simulink model "Main_SpeedOptimisedVersionTannenweg"  (R2024b)
settings: Solver=ode15s  StartTime=0.0  StopTime=3600*2  FixedStep=0.1  RelTol=0.001
model workspace (MAT data in the model file):
  Ti = 5
  fa = 0.00071
  fd = 0.03
  ips = 36
  ma = 0.0013
  md = 0.04
  roomarea1 = 20
  s = 15
libraries: fl_lib x1434, nesl_utility x105, SimscapeFluids_lib x35
(part 2 of 22)

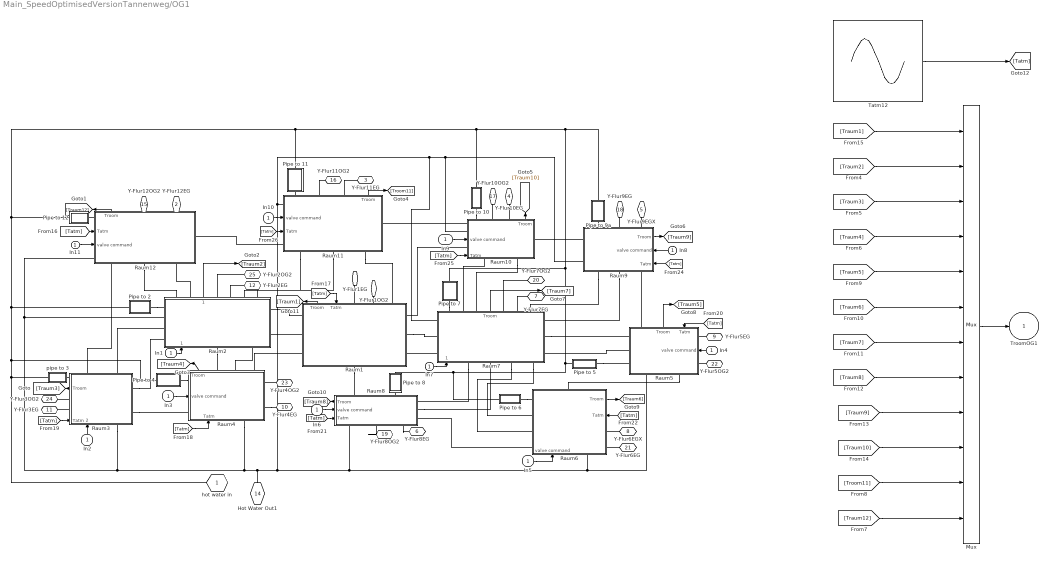
== system Main_SpeedOptimisedVersionTannenweg/OG1 ==
  In1 : Inport
  In{2..11} (10 alike) : InportShadow
  Mux : Mux  Inputs=12
  Pipe to 10 : Subsystem
  Pipe to 11 : Subsystem
  Pipe to 12 : Subsystem
  Pipe to 2 : Subsystem
  Pipe to 4 : Subsystem
  Pipe to 5 : Subsystem
  Pipe to 6 : Subsystem
  Pipe to 7 : Subsystem
  Pipe to 8 : Subsystem
  Pipe to 9a : Subsystem
  Raum1 : Subsystem
      settings: PortSchema="{\"entries\":[{\"content\":{\"sides\":[{\"content\":{\"connectorIds\":[\"LConn1\",\"LConn2\",\"LConn3\"]},\"type\":\"ConnectorPlacement.EquallySpacedRectSide\",\"uuid\":\"258852ae-79b4-4e90-ae22-4154c858ab0a\"},{\"content\":{\"connectorIds\":[\"RConn1\",\"RConn2\",\"RConn3\"],\"side\":\"RIGHT\"},\"type\":\"ConnectorPlacement.EquallySpacedRectSide\",\"uuid\":\"36706832-f330-42ce-9a32-f145cdee4912\"},{\"content\":{\"connectorIds\":[\"LConn4\",\"LConn5\",\"LConn6\",\"In1\",\"Out1\"],\"side\":\"TOP\"},\"type\":\"ConnectorPlacement.EquallySpacedRectSide\",\"uuid\":\"5cf2347a-3520-447e-9561-2d1c8313f3cf\"},{\"content\":{\"connectorIds\":[\"RConn4\"],\"side\":\"BOTTOM\"},\"type\":\"ConnectorPlacement.EquallySpacedRectSide\",\"uuid\":\"b1588268-8d41-4423-8f6e-2c28bf9b13dc\"}]},\"type\":\"ConnectorPlacement.EquallySpacedConnector\",\"uuid\":\"6bed35e7-1d7a-421b-a1f8-39267ed9017d\"}],\"packageUris\":[\"http://schema.mathworks.com/mf0/Connector/R2020b\"],\"version\":\"1.0\"}"
  Raum10 : Subsystem
      settings: PortSchema="{\"entries\":[{\"content\":{\"sides\":[{\"content\":{\"connectorIds\":[\"LConn1\",\"LConn2\",\"In1\",\"LConn3\",\"In2\"]},\"type\":\"ConnectorPlacement.EquallySpacedRectSide\",\"uuid\":\"258852ae-79b4-4e90-ae22-4154c858ab0a\"},{\"content\":{\"connectorIds\":[\"RConn1\"],\"side\":\"RIGHT\"},\"type\":\"ConnectorPlacement.EquallySpacedRectSide\",\"uuid\":\"36706832-f330-42ce-9a32-f145cdee4912\"},{\"content\":{\"connectorIds\":[\"LConn4\",\"LConn5\",\"LConn6\",\"Out1\"],\"side\":\"TOP\"},\"type\":\"ConnectorPlacement.EquallySpacedRectSide\",\"uuid\":\"5cf2347a-3520-447e-9561-2d1c8313f3cf\"},{\"content\":{\"connectorIds\":[\"RConn2\",\"RConn3\"],\"side\":\"BOTTOM\"},\"type\":\"ConnectorPlacement.EquallySpacedRectSide\",\"uuid\":\"b1588268-8d41-4423-8f6e-2c28bf9b13dc\"}]},\"type\":\"ConnectorPlacement.EquallySpacedConnector\",\"uuid\":\"6bed35e7-1d7a-421b-a1f8-39267ed9017d\"}],\"packageUris\":[\"http://schema.mathworks.com/mf0/Connector/R2020b\"],\"version\":\"1.0\"}"
  Raum11 : Subsystem
      settings: PortSchema="{\"entries\":[{\"content\":{\"sides\":[{\"content\":{\"connectorIds\":[\"LConn1\",\"In1\",\"In2\",\"LConn2\"]},\"type\":\"ConnectorPlacement.EquallySpacedRectSide\",\"uuid\":\"258852ae-79b4-4e90-ae22-4154c858ab0a\"},{\"content\":{\"connectorIds\":[\"RConn1\"],\"side\":\"RIGHT\"},\"type\":\"ConnectorPlacement.EquallySpacedRectSide\",\"uuid\":\"36706832-f330-42ce-9a32-f145cdee4912\"},{\"content\":{\"connectorIds\":[\"LConn3\",\"LConn4\",\"LConn5\",\"Out1\"],\"side\":\"TOP\"},\"type\":\"ConnectorPlacement.EquallySpacedRectSide\",\"uuid\":\"5cf2347a-3520-447e-9561-2d1c8313f3cf\"},{\"content\":{\"connectorIds\":[\"RConn2\",\"RConn3\",\"RConn4\"],\"side\":\"BOTTOM\"},\"type\":\"ConnectorPlacement.EquallySpacedRectSide\",\"uuid\":\"b1588268-8d41-4423-8f6e-2c28bf9b13dc\"}]},\"type\":\"ConnectorPlacement.EquallySpacedConnector\",\"uuid\":\"6bed35e7-1d7a-421b-a1f8-39267ed9017d\"}],\"packageUris\":[\"http://schema.mathworks.com/mf0/Connector/R2020b\"],\"version\":\"1.0\"}"
  Raum12 : Subsystem
      settings: PortSchema="{\"entries\":[{\"content\":{\"sides\":[{\"content\":{\"connectorIds\":[\"LConn1\",\"In1\",\"In2\",\"LConn2\"]},\"type\":\"ConnectorPlacement.EquallySpacedRectSide\",\"uuid\":\"258852ae-79b4-4e90-ae22-4154c858ab0a\"},{\"content\":{\"connectorIds\":[\"RConn1\"],\"side\":\"RIGHT\"},\"type\":\"ConnectorPlacement.EquallySpacedRectSide\",\"uuid\":\"36706832-f330-42ce-9a32-f145cdee4912\"},{\"content\":{\"connectorIds\":[\"Out1\",\"LConn3\",\"LConn4\"],\"side\":\"TOP\"},\"type\":\"ConnectorPlacement.EquallySpacedRectSide\",\"uuid\":\"5cf2347a-3520-447e-9561-2d1c8313f3cf\"},{\"content\":{\"connectorIds\":[\"RConn2\",\"RConn3\",\"RConn4\"],\"side\":\"BOTTOM\"},\"type\":\"ConnectorPlacement.EquallySpacedRectSide\",\"uuid\":\"b1588268-8d41-4423-8f6e-2c28bf9b13dc\"}]},\"type\":\"ConnectorPlacement.EquallySpacedConnector\",\"uuid\":\"6bed35e7-1d7a-421b-a1f8-39267ed9017d\"}],\"packageUris\":[\"http://schema.mathworks.com/mf0/Connector/R2020b\"],\"version\":\"1.0\"}"
  Raum2 : Subsystem
      settings: PortSchema="{\"entries\":[{\"content\":{\"sides\":[{\"content\":{\"connectorIds\":[\"LConn1\",\"LConn2\",\"LConn3\",\"LConn4\"]},\"type\":\"ConnectorPlacement.EquallySpacedRectSide\",\"uuid\":\"258852ae-79b4-4e90-ae22-4154c858ab0a\"},{\"content\":{\"connectorIds\":[\"RConn1\",\"RConn2\"],\"side\":\"RIGHT\"},\"type\":\"ConnectorPlacement.EquallySpacedRectSide\",\"uuid\":\"36706832-f330-42ce-9a32-f145cdee4912\"},{\"content\":{\"connectorIds\":[\"LConn5\",\"LConn6\",\"Out1\",\"LConn7\",\"LConn8\",\"LConn9\",\"LConn10\"],\"side\":\"TOP\"},\"type\":\"ConnectorPlacement.EquallySpacedRectSide\",\"uuid\":\"5cf2347a-3520-447e-9561-2d1c8313f3cf\"},{\"content\":{\"connectorIds\":[\"In1\",\"RConn3\",\"RConn4\"],\"side\":\"BOTTOM\"},\"type\":\"ConnectorPlacement.EquallySpacedRectSide\",\"uuid\":\"b1588268-8d41-4423-8f6e-2c28bf9b13dc\"}]},\"type\":\"ConnectorPlacement.EquallySpacedConnector\",\"uuid\":\"6bed35e7-1d7a-421b-a1f8-39267ed9017d\"}],\"packageUris\":[\"http://schema.mathworks.com/mf0/Connector/R2020b\"],\"version\":\"1.0\"}"
  Raum3 : Subsystem
      settings: PortSchema="{\"entries\":[{\"content\":{\"sides\":[{\"content\":{\"connectorIds\":[\"LConn1\",\"Out1\",\"LConn2\",\"LConn3\",\"In1\"]},\"type\":\"ConnectorPlacement.EquallySpacedRectSide\",\"uuid\":\"258852ae-79b4-4e90-ae22-4154c858ab0a\"},{\"content\":{\"connectorIds\":[\"RConn1\",\"RConn2\"],\"side\":\"RIGHT\"},\"type\":\"ConnectorPlacement.EquallySpacedRectSide\",\"uuid\":\"36706832-f330-42ce-9a32-f145cdee4912\"},{\"content\":{\"connectorIds\":[\"LConn4\",\"LConn5\"],\"side\":\"TOP\"},\"type\":\"ConnectorPlacement.EquallySpacedRectSide\",\"uuid\":\"5cf2347a-3520-447e-9561-2d1c8313f3cf\"},{\"content\":{\"connectorIds\":[\"In2\",\"RConn3\"],\"side\":\"BOTTOM\"},\"type\":\"ConnectorPlacement.EquallySpacedRectSide\",\"uuid\":\"b1588268-8d41-4423-8f6e-2c28bf9b13dc\"}]},\"type\":\"ConnectorPlacement.EquallySpacedConnector\",\"uuid\":\"6bed35e7-1d7a-421b-a1f8-39267ed9017d\"}],\"packageUris\":[\"http://schema.mathworks.com/mf0/Connector/R2020b\"],\"version\":\"1.0\"}"
  Raum4 : Subsystem
      settings: PortSchema="{\"entries\":[{\"content\":{\"sides\":[{\"content\":{\"connectorIds\":[\"LConn1\",\"In1\",\"LConn2\"]},\"type\":\"ConnectorPlacement.EquallySpacedRectSide\",\"uuid\":\"258852ae-79b4-4e90-ae22-4154c858ab0a\"},{\"content\":{\"connectorIds\":[\"RConn1\",\"RConn2\"],\"side\":\"RIGHT\"},\"type\":\"ConnectorPlacement.EquallySpacedRectSide\",\"uuid\":\"36706832-f330-42ce-9a32-f145cdee4912\"},{\"content\":{\"connectorIds\":[\"Out1\",\"LConn3\",\"LConn4\",\"LConn5\"],\"side\":\"TOP\"},\"type\":\"ConnectorPlacement.EquallySpacedRectSide\",\"uuid\":\"5cf2347a-3520-447e-9561-2d1c8313f3cf\"},{\"content\":{\"connectorIds\":[\"In2\",\"RConn3\"],\"side\":\"BOTTOM\"},\"type\":\"ConnectorPlacement.EquallySpacedRectSide\",\"uuid\":\"b1588268-8d41-4423-8f6e-2c28bf9b13dc\"}]},\"type\":\"ConnectorPlacement.EquallySpacedConnector\",\"uuid\":\"6bed35e7-1d7a-421b-a1f8-39267ed9017d\"}],\"packageUris\":[\"http://schema.mathworks.com/mf0/Connector/R2020b\"],\"version\":\"1.0\"}"
  Raum5 : Subsystem
      settings: PortSchema="{\"entries\":[{\"content\":{\"sides\":[{\"content\":{\"connectorIds\":[\"LConn1\",\"LConn2\",\"LConn3\"]},\"type\":\"ConnectorPlacement.EquallySpacedRectSide\",\"uuid\":\"258852ae-79b4-4e90-ae22-4154c858ab0a\"},{\"content\":{\"connectorIds\":[\"RConn1\",\"In2\",\"RConn2\"],\"side\":\"RIGHT\"},\"type\":\"ConnectorPlacement.EquallySpacedRectSide\",\"uuid\":\"36706832-f330-42ce-9a32-f145cdee4912\"},{\"content\":{\"connectorIds\":[\"LConn4\",\"Out1\",\"In1\"],\"side\":\"TOP\"},\"type\":\"ConnectorPlacement.EquallySpacedRectSide\",\"uuid\":\"5cf2347a-3520-447e-9561-2d1c8313f3cf\"},{\"content\":{\"connectorIds\":[\"RConn3\",\"RConn4\"],\"side\":\"BOTTOM\"},\"type\":\"ConnectorPlacement.EquallySpacedRectSide\",\"uuid\":\"b1588268-8d41-4423-8f6e-2c28bf9b13dc\"}]},\"type\":\"ConnectorPlacement.EquallySpacedConnector\",\"uuid\":\"6bed35e7-1d7a-421b-a1f8-39267ed9017d\"}],\"packageUris\":[\"http://schema.mathworks.com/mf0/Connector/R2020b\"],\"version\":\"1.0\"}"
  Raum6 : Subsystem
      settings: PortSchema="{\"entries\":[{\"content\":{\"sides\":[{\"content\":{\"connectorIds\":[\"LConn1\",\"LConn2\",\"LConn3\",\"LConn4\"]},\"type\":\"ConnectorPlacement.EquallySpacedRectSide\",\"uuid\":\"258852ae-79b4-4e90-ae22-4154c858ab0a\"},{\"content\":{\"connectorIds\":[\"Out1\",\"In2\",\"RConn1\",\"RConn2\"],\"side\":\"RIGHT\"},\"type\":\"ConnectorPlacement.EquallySpacedRectSide\",\"uuid\":\"36706832-f330-42ce-9a32-f145cdee4912\"},{\"content\":{\"connectorIds\":[\"LConn5\"],\"side\":\"TOP\"},\"type\":\"ConnectorPlacement.EquallySpacedRectSide\",\"uuid\":\"5cf2347a-3520-447e-9561-2d1c8313f3cf\"},{\"content\":{\"connectorIds\":[\"In1\",\"RConn3\"],\"side\":\"BOTTOM\"},\"type\":\"ConnectorPlacement.EquallySpacedRectSide\",\"uuid\":\"b1588268-8d41-4423-8f6e-2c28bf9b13dc\"}]},\"type\":\"ConnectorPlacement.EquallySpacedConnector\",\"uuid\":\"6bed35e7-1d7a-421b-a1f8-39267ed9017d\"}],\"packageUris\":[\"http://schema.mathworks.com/mf0/Connector/R2020b\"],\"version\":\"1.0\"}"
  Raum7 : Subsystem
      settings: PortSchema="{\"entries\":[{\"content\":{\"sides\":[{\"content\":{\"connectorIds\":[\"LConn1\",\"LConn2\",\"LConn3\"]},\"type\":\"ConnectorPlacement.EquallySpacedRectSide\",\"uuid\":\"258852ae-79b4-4e90-ae22-4154c858ab0a\"},{\"content\":{\"connectorIds\":[\"RConn1\",\"RConn2\",\"RConn3\"],\"side\":\"RIGHT\"},\"type\":\"ConnectorPlacement.EquallySpacedRectSide\",\"uuid\":\"36706832-f330-42ce-9a32-f145cdee4912\"},{\"content\":{\"connectorIds\":[\"LConn4\",\"LConn5\",\"LConn6\",\"Out1\",\"LConn7\",\"LConn8\",\"LConn9\"],\"side\":\"TOP\"},\"type\":\"ConnectorPlacement.EquallySpacedRectSide\",\"uuid\":\"5cf2347a-3520-447e-9561-2d1c8313f3cf\"},{\"content\":{\"connectorIds\":[\"In1\",\"RConn4\",\"RConn5\",\"RConn6\",\"RConn7\"],\"side\":\"BOTTOM\"},\"type\":\"ConnectorPlacement.EquallySpacedRectSide\",\"uuid\":\"b1588268-8d41-4423-8f6e-2c28bf9b13dc\"}]},\"type\":\"ConnectorPlacement.EquallySpacedConnector\",\"uuid\":\"6bed35e7-1d7a-421b-a1f8-39267ed9017d\"}],\"packageUris\":[\"http://schema.mathworks.com/mf0/Connector/R2020b\"],\"version\":\"1.0\"}"
  Raum8 : Subsystem
      settings: PortSchema="{\"entries\":[{\"content\":{\"sides\":[{\"content\":{\"connectorIds\":[\"Out1\",\"In1\",\"In2\"]},\"type\":\"ConnectorPlacement.EquallySpacedRectSide\",\"uuid\":\"258852ae-79b4-4e90-ae22-4154c858ab0a\"},{\"content\":{\"connectorIds\":[\"RConn1\",\"RConn2\",\"RConn3\"],\"side\":\"RIGHT\"},\"type\":\"ConnectorPlacement.EquallySpacedRectSide\",\"uuid\":\"36706832-f330-42ce-9a32-f145cdee4912\"},{\"content\":{\"connectorIds\":[\"LConn1\",\"LConn2\"],\"side\":\"TOP\"},\"type\":\"ConnectorPlacement.EquallySpacedRectSide\",\"uuid\":\"5cf2347a-3520-447e-9561-2d1c8313f3cf\"},{\"content\":{\"connectorIds\":[\"RConn4\",\"RConn5\",\"RConn6\"],\"side\":\"BOTTOM\"},\"type\":\"ConnectorPlacement.EquallySpacedRectSide\",\"uuid\":\"b1588268-8d41-4423-8f6e-2c28bf9b13dc\"}]},\"type\":\"ConnectorPlacement.EquallySpacedConnector\",\"uuid\":\"6bed35e7-1d7a-421b-a1f8-39267ed9017d\"}],\"packageUris\":[\"http://schema.mathworks.com/mf0/Connector/R2020b\"],\"version\":\"1.0\"}"
  Raum9 : Subsystem
      settings: PortSchema="{\"entries\":[{\"content\":{\"sides\":[{\"content\":{\"connectorIds\":[\"LConn1\",\"LConn2\"]},\"type\":\"ConnectorPlacement.EquallySpacedRectSide\",\"uuid\":\"258852ae-79b4-4e90-ae22-4154c858ab0a\"},{\"content\":{\"connectorIds\":[\"Out1\",\"In1\",\"In2\"],\"side\":\"RIGHT\"},\"type\":\"ConnectorPlacement.EquallySpacedRectSide\",\"uuid\":\"36706832-f330-42ce-9a32-f145cdee4912\"},{\"content\":{\"connectorIds\":[\"LConn3\",\"LConn4\",\"LConn5\"],\"side\":\"TOP\"},\"type\":\"ConnectorPlacement.EquallySpacedRectSide\",\"uuid\":\"5cf2347a-3520-447e-9561-2d1c8313f3cf\"},{\"content\":{\"connectorIds\":[\"RConn1\",\"RConn2\",\"RConn3\"],\"side\":\"BOTTOM\"},\"type\":\"ConnectorPlacement.EquallySpacedRectSide\",\"uuid\":\"b1588268-8d41-4423-8f6e-2c28bf9b13dc\"}]},\"type\":\"ConnectorPlacement.EquallySpacedConnector\",\"uuid\":\"6bed35e7-1d7a-421b-a1f8-39267ed9017d\"}],\"packageUris\":[\"http://schema.mathworks.com/mf0/Connector/R2020b\"],\"version\":\"1.0\"}"
  Tatm12 : Sin  Amplitude=7  Frequency=2*pi/(24*3600)  Phase=pi  SampleTime=0
  pipe to 3 : Subsystem
  hot water in : PMIOPort  Side=Left
  Y-Flur12EG : PMIOPort  Port=2  Side=Left
  Y-Flur11EG : PMIOPort  Port=3  Side=Left
  Y-Flur10EG : PMIOPort  Port=4  Side=Left
  Y-Flur9EGX : PMIOPort  Port=5  Side=Left
  Y-Flur8EG : PMIOPort  Port=6  Side=Left
  Y-Flur7EG : PMIOPort  Port=7  Side=Left
  Y-Flur6EGX : PMIOPort  Port=8  Side=Left
  Y-Flur5EG : PMIOPort  Port=9  Side=Left
  Y-Flur4EG : PMIOPort  Port=10  Side=Left
  Y-Flur3EG : PMIOPort  Port=11  Side=Left
  Y-Flur2EG : PMIOPort  Port=12  Side=Left
  Y-Flur1EG : PMIOPort  Port=13  Side=Left
  Hot Water Out1 : PMIOPort  Port=14  Side=Right
  Y-Flur12OG2 : PMIOPort  Port=15  Side=Right
  Y-Flur11OG2 : PMIOPort  Port=16  Side=Right
  Y-Flur10OG2 : PMIOPort  Port=17  Side=Right
  Y-Flur9EG : PMIOPort  Port=18  Side=Right
  Y-Flur8OG2 : PMIOPort  Port=19  Side=Right
  Y-Flur7OG2 : PMIOPort  Port=20  Side=Right
  Y-Flur6EG : PMIOPort  Port=21  Side=Right
  Y-Flur5OG2 : PMIOPort  Port=22  Side=Right
  Y-Flur4OG2 : PMIOPort  Port=23  Side=Right
  Y-Flur3OG2 : PMIOPort  Port=24  Side=Right
  Y-Flur2OG2 : PMIOPort  Port=25  Side=Right
  Y-Flur1OG2 : PMIOPort  Port=26  Side=Right
  TroomOG1 : Outport
  wires:
  [Tatm] -> Raum12/1(Tatm)
  Raum12/1(Troom) -> [Traum12]
  Raum8/1(Troom) -> [Traum8]
  Raum5/1(Troom) -> [Traum5]
  Raum4/1(Troom) -> [Traum4]
  [Tatm] -> Raum8/2(Tatm)
  [Tatm] -> Raum6/2(Tatm)
  Raum1/1(Troom) -> [Traum1]
  Raum10/1(Troom) -> [Traum10]
  Raum3/1(Troom) -> [Traum3]
  [Tatm] -> Raum4/2(Tatm)
  [Tatm] -> Raum3/1(Tatm)
  [Tatm] -> Raum5/1(Tatm)
  [Tatm] -> Raum1/1(Tatm)
  [Tatm] -> Raum10/2(Tatm)
  Raum2/1(Troom) -> [Traum2]
  Raum11/1(Troom) -> [Troom11]
  Raum7/1(Troom) -> [Traum7]
  [Tatm] -> Raum9/2(Tatm)
  Raum6/1(Troom) -> [Traum6]
  [Tatm] -> Raum11/2(Tatm)
  Raum9/1(Troom) -> [Traum9]
  Tatm12/1 -> [Tatm]
  In1/1 -> Raum2/1(valve command)
  In2/1 -> Raum3/2(valve command)
  In3/1 -> Raum4/1(valve command)
  In6/1 -> Raum8/1(valve command)
  In5/1 -> Raum6/1(valve command)
  In4/1 -> Raum5/2(valve command)
  In7/1 -> Raum7/1(valve command)
  In8/1 -> Raum9/1(valve command)
  In9/1 -> Raum10/1(valve command)
  In10/1 -> Raum11/1(valve command)
  In11/1 -> Raum12/2(valve command)
  [Traum9] -> Mux/9
  [Traum7] -> Mux/7
  [Traum8] -> Mux/8
  [Traum12] -> Mux/12
  [Traum5] -> Mux/5
  [Traum6] -> Mux/6
  [Traum3] -> Mux/3
  [Traum4] -> Mux/4
  Mux/1 -> TroomOG1/1
  [Traum2] -> Mux/2
  [Traum1] -> Mux/1
  [Troom11] -> Mux/11
  [Traum10] -> Mux/10
  connections:
  Raum2/LConn7 -- Y-Flur2OG2/RConn1
  Raum3/LConn2 -- Y-Flur3OG2/RConn1
  Y-Flur4OG2/RConn1 -- Raum4/RConn1
  Raum1/LConn5 -- Y-Flur1OG2/RConn1
  Y-Flur8OG2/RConn1 -- Raum8/RConn5
  Y-Flur6EG/RConn1 -- Raum6/RConn2
  Raum7/LConn7 -- Y-Flur7OG2/RConn1
  Y-Flur5OG2/RConn1 -- Raum5/RConn2
  Raum9/LConn4 -- Y-Flur9EG/RConn1
  Raum10/LConn5 -- Y-Flur10OG2/RConn1
  Raum11/LConn4 -- Y-Flur11OG2/RConn1
  Raum12/LConn3 -- Y-Flur12OG2/RConn1
  Raum2/RConn1 -- Raum1/RConn1
  Raum7/LConn5 -- Raum10/RConn2
  Raum8/RConn2 -- Raum7/RConn5
  Raum11/RConn3 -- Raum2/LConn10
  Raum1/LConn2 -- Raum7/LConn2
  Raum1/RConn3 -- Raum4/LConn5
  Pipe to 5/RConn1 -- Raum5/LConn3
  Raum3/RConn2 -- Raum4/LConn2
  Raum9/RConn1 -- Raum7/LConn9
  Raum3/RConn1 -- Raum2/LConn4
  Raum11/RConn2 -- Raum2/LConn9
  Raum7/RConn2 -- Raum5/LConn1
  Raum10/RConn3 -- Raum7/LConn6
  Raum12/RConn3 -- Raum2/LConn5
  Pipe to 2/RConn1 -- Raum2/LConn1
  Raum10/LConn3 -- Raum1/LConn1
  Raum3/LConn4 -- Raum12/RConn2
  Raum7/RConn4 -- Raum8/RConn1
  Raum2/RConn3 -- Raum4/LConn3
  Raum5/LConn2 -- Raum7/RConn3
  Raum9/LConn1 -- Raum10/RConn1
  Raum1/RConn4 -- Raum8/LConn1
  pipe to 3/RConn1 -- Raum3/LConn1
  Pipe to 10/RConn1 -- Raum10/LConn4
  Raum7/LConn3 -- Raum1/LConn3
  Raum2/LConn6 -- Raum12/RConn4
  Raum10/LConn1 -- Raum11/RConn1
  Raum9/RConn2 -- Raum7/RConn1
  Pipe to 11/RConn1 -- Raum11/LConn3
  Pipe to 8/RConn1 -- Raum8/LConn2
  Raum7/RConn7 -- Raum6/LConn2
  Pipe to 4/RConn1 -- Raum4/LConn1
  Raum5/LConn4 -- Raum9/RConn3
  Raum9/LConn3 -- Pipe to 9a/RConn1
  Raum11/RConn4 -- Raum1/LConn4
  Raum4/LConn4 -- Raum2/RConn4
  Raum3/LConn5 -- Raum2/LConn3
  Raum11/LConn2 -- Raum12/RConn1
  Pipe to 7/RConn1 -- Raum7/LConn4
  Pipe to 12/RConn1 -- Raum12/LConn1
  Raum1/RConn2 -- Raum2/RConn2
  Pipe to 6/RConn1 -- Raum6/LConn1
  Raum7/RConn6 -- Raum6/LConn3
  Raum5/RConn4 -- Raum6/LConn5
  Raum11/LConn1 -- Raum9/LConn2 -- Raum10/LConn2 -- Raum7/LConn1 -- Raum4/RConn3 -- Raum3/RConn3 -- Raum2/LConn2 -- Raum12/LConn2 -- Hot Water Out1/RConn1 -- Raum5/RConn3 -- Raum6/RConn3 -- Raum8/RConn4
  Raum6/LConn4 -- Raum8/RConn3
  Raum1/LConn6 -- Y-Flur1EG/RConn1
  Raum3/LConn3 -- Y-Flur3EG/RConn1
  Raum4/RConn2 -- Y-Flur4EG/RConn1
  Y-Flur5EG/RConn1 -- Raum5/RConn1
  Y-Flur6EGX/RConn1 -- Raum6/RConn1
  Raum7/LConn8 -- Y-Flur7EG/RConn1
  Raum8/RConn6 -- Y-Flur8EG/RConn1
  Raum9/LConn5 -- Y-Flur9EGX/RConn1
  Raum10/LConn6 -- Y-Flur10EG/RConn1
  Raum11/LConn5 -- Y-Flur11EG/RConn1
  Raum12/LConn4 -- Y-Flur12EG/RConn1
  Raum2/LConn8 -- Y-Flur2EG/RConn1
  Pipe to 9a/LConn1 -- hot water in/RConn1 -- pipe to 3/LConn1 -- Pipe to 4/LConn1 -- Pipe to 2/LConn1 -- Pipe to 12/LConn1 -- Pipe to 11/LConn1 -- Pipe to 10/LConn1 -- Pipe to 6/LConn1 -- Pipe to 8/LConn1 -- Pipe to 5/LConn1 -- Pipe to 7/LConn1

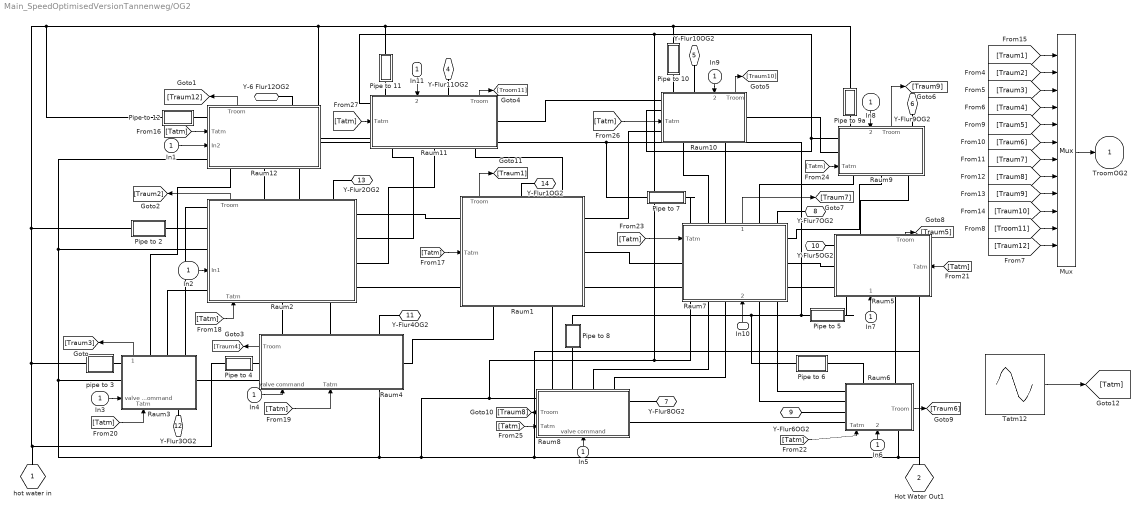
== system Main_SpeedOptimisedVersionTannenweg/OG2 ==
  In1 : Inport
  In{2..11} (10 alike) : InportShadow
  Mux : Mux  Inputs=12
  Pipe to 10 : Subsystem
  Pipe to 11 : Subsystem
  Pipe to 12 : Subsystem
  Pipe to 2 : Subsystem
  Pipe to 4 : Subsystem
  Pipe to 5 : Subsystem
  Pipe to 6 : Subsystem
  Pipe to 7 : Subsystem
  Pipe to 8 : Subsystem
  Pipe to 9a : Subsystem
  Raum1 : Subsystem
      settings: PortSchema="{\"entries\":[{\"content\":{\"sides\":[{\"content\":{\"connectorIds\":[\"LConn1\",\"LConn2\",\"LConn3\"]},\"type\":\"ConnectorPlacement.EquallySpacedRectSide\",\"uuid\":\"258852ae-79b4-4e90-ae22-4154c858ab0a\"},{\"content\":{\"connectorIds\":[\"RConn1\",\"In1\",\"RConn2\"],\"side\":\"RIGHT\"},\"type\":\"ConnectorPlacement.EquallySpacedRectSide\",\"uuid\":\"36706832-f330-42ce-9a32-f145cdee4912\"},{\"content\":{\"connectorIds\":[\"LConn4\",\"LConn5\",\"Out1\"],\"side\":\"TOP\"},\"type\":\"ConnectorPlacement.EquallySpacedRectSide\",\"uuid\":\"5cf2347a-3520-447e-9561-2d1c8313f3cf\"},{\"content\":{\"connectorIds\":[\"RConn3\",\"RConn4\"],\"side\":\"BOTTOM\"},\"type\":\"ConnectorPlacement.EquallySpacedRectSide\",\"uuid\":\"b1588268-8d41-4423-8f6e-2c28bf9b13dc\"}]},\"type\":\"ConnectorPlacement.EquallySpacedConnector\",\"uuid\":\"6bed35e7-1d7a-421b-a1f8-39267ed9017d\"}],\"packageUris\":[\"http://schema.mathworks.com/mf0/Connector/R2020b\"],\"version\":\"1.0\"}"
  Raum10 : Subsystem
      settings: PortSchema="{\"entries\":[{\"content\":{\"sides\":[{\"content\":{\"connectorIds\":[\"LConn1\",\"LConn2\",\"In1\",\"LConn3\"]},\"type\":\"ConnectorPlacement.EquallySpacedRectSide\",\"uuid\":\"258852ae-79b4-4e90-ae22-4154c858ab0a\"},{\"content\":{\"connectorIds\":[\"RConn1\"],\"side\":\"RIGHT\"},\"type\":\"ConnectorPlacement.EquallySpacedRectSide\",\"uuid\":\"36706832-f330-42ce-9a32-f145cdee4912\"},{\"content\":{\"connectorIds\":[\"LConn4\",\"LConn5\",\"In2\",\"Out1\"],\"side\":\"TOP\"},\"type\":\"ConnectorPlacement.EquallySpacedRectSide\",\"uuid\":\"5cf2347a-3520-447e-9561-2d1c8313f3cf\"},{\"content\":{\"connectorIds\":[\"RConn2\",\"RConn3\"],\"side\":\"BOTTOM\"},\"type\":\"ConnectorPlacement.EquallySpacedRectSide\",\"uuid\":\"b1588268-8d41-4423-8f6e-2c28bf9b13dc\"}]},\"type\":\"ConnectorPlacement.EquallySpacedConnector\",\"uuid\":\"6bed35e7-1d7a-421b-a1f8-39267ed9017d\"}],\"packageUris\":[\"http://schema.mathworks.com/mf0/Connector/R2020b\"],\"version\":\"1.0\"}"
  Raum11 : Subsystem
      settings: PortSchema="{\"entries\":[{\"content\":{\"sides\":[{\"content\":{\"connectorIds\":[\"LConn1\",\"In1\",\"LConn2\"]},\"type\":\"ConnectorPlacement.EquallySpacedRectSide\",\"uuid\":\"258852ae-79b4-4e90-ae22-4154c858ab0a\"},{\"content\":{\"connectorIds\":[\"RConn1\"],\"side\":\"RIGHT\"},\"type\":\"ConnectorPlacement.EquallySpacedRectSide\",\"uuid\":\"36706832-f330-42ce-9a32-f145cdee4912\"},{\"content\":{\"connectorIds\":[\"LConn3\",\"In2\",\"LConn4\",\"Out1\"],\"side\":\"TOP\"},\"type\":\"ConnectorPlacement.EquallySpacedRectSide\",\"uuid\":\"5cf2347a-3520-447e-9561-2d1c8313f3cf\"},{\"content\":{\"connectorIds\":[\"RConn2\",\"RConn3\",\"RConn4\"],\"side\":\"BOTTOM\"},\"type\":\"ConnectorPlacement.EquallySpacedRectSide\",\"uuid\":\"b1588268-8d41-4423-8f6e-2c28bf9b13dc\"}]},\"type\":\"ConnectorPlacement.EquallySpacedConnector\",\"uuid\":\"6bed35e7-1d7a-421b-a1f8-39267ed9017d\"}],\"packageUris\":[\"http://schema.mathworks.com/mf0/Connector/R2020b\"],\"version\":\"1.0\"}"
  Raum12 : Subsystem
      settings: PortSchema="{\"entries\":[{\"content\":{\"sides\":[{\"content\":{\"connectorIds\":[\"LConn1\",\"In1\",\"In2\",\"LConn2\"]},\"type\":\"ConnectorPlacement.EquallySpacedRectSide\",\"uuid\":\"258852ae-79b4-4e90-ae22-4154c858ab0a\"},{\"content\":{\"connectorIds\":[\"RConn1\"],\"side\":\"RIGHT\"},\"type\":\"ConnectorPlacement.EquallySpacedRectSide\",\"uuid\":\"36706832-f330-42ce-9a32-f145cdee4912\"},{\"content\":{\"connectorIds\":[\"Out1\",\"LConn3\"],\"side\":\"TOP\"},\"type\":\"ConnectorPlacement.EquallySpacedRectSide\",\"uuid\":\"5cf2347a-3520-447e-9561-2d1c8313f3cf\"},{\"content\":{\"connectorIds\":[\"RConn2\",\"RConn3\",\"RConn4\"],\"side\":\"BOTTOM\"},\"type\":\"ConnectorPlacement.EquallySpacedRectSide\",\"uuid\":\"b1588268-8d41-4423-8f6e-2c28bf9b13dc\"}]},\"type\":\"ConnectorPlacement.EquallySpacedConnector\",\"uuid\":\"6bed35e7-1d7a-421b-a1f8-39267ed9017d\"}],\"packageUris\":[\"http://schema.mathworks.com/mf0/Connector/R2020b\"],\"version\":\"1.0\"}"
  Raum2 : Subsystem
      settings: PortSchema="{\"entries\":[{\"content\":{\"sides\":[{\"content\":{\"connectorIds\":[\"LConn1\",\"LConn2\",\"LConn3\",\"In1\",\"LConn4\"]},\"type\":\"ConnectorPlacement.EquallySpacedRectSide\",\"uuid\":\"258852ae-79b4-4e90-ae22-4154c858ab0a\"},{\"content\":{\"connectorIds\":[\"RConn1\",\"RConn2\",\"RConn3\",\"RConn4\"],\"side\":\"RIGHT\"},\"type\":\"ConnectorPlacement.EquallySpacedRectSide\",\"uuid\":\"36706832-f330-42ce-9a32-f145cdee4912\"},{\"content\":{\"connectorIds\":[\"Out1\",\"LConn5\",\"LConn6\",\"LConn7\"],\"side\":\"TOP\"},\"type\":\"ConnectorPlacement.EquallySpacedRectSide\",\"uuid\":\"5cf2347a-3520-447e-9561-2d1c8313f3cf\"},{\"content\":{\"connectorIds\":[\"In2\",\"RConn5\",\"RConn6\"],\"side\":\"BOTTOM\"},\"type\":\"ConnectorPlacement.EquallySpacedRectSide\",\"uuid\":\"b1588268-8d41-4423-8f6e-2c28bf9b13dc\"}]},\"type\":\"ConnectorPlacement.EquallySpacedConnector\",\"uuid\":\"6bed35e7-1d7a-421b-a1f8-39267ed9017d\"}],\"packageUris\":[\"http://schema.mathworks.com/mf0/Connector/R2020b\"],\"version\":\"1.0\"}"
  Raum3 : Subsystem
      settings: PortSchema="{\"entries\":[{\"content\":{\"sides\":[{\"content\":{\"connectorIds\":[\"LConn1\",\"LConn2\",\"In1\"]},\"type\":\"ConnectorPlacement.EquallySpacedRectSide\",\"uuid\":\"258852ae-79b4-4e90-ae22-4154c858ab0a\"},{\"content\":{\"connectorIds\":[\"RConn1\"],\"side\":\"RIGHT\"},\"type\":\"ConnectorPlacement.EquallySpacedRectSide\",\"uuid\":\"36706832-f330-42ce-9a32-f145cdee4912\"},{\"content\":{\"connectorIds\":[\"Out1\",\"LConn3\",\"LConn4\",\"LConn5\"],\"side\":\"TOP\"},\"type\":\"ConnectorPlacement.EquallySpacedRectSide\",\"uuid\":\"5cf2347a-3520-447e-9561-2d1c8313f3cf\"},{\"content\":{\"connectorIds\":[\"In2\",\"RConn2\"],\"side\":\"BOTTOM\"},\"type\":\"ConnectorPlacement.EquallySpacedRectSide\",\"uuid\":\"b1588268-8d41-4423-8f6e-2c28bf9b13dc\"}]},\"type\":\"ConnectorPlacement.EquallySpacedConnector\",\"uuid\":\"6bed35e7-1d7a-421b-a1f8-39267ed9017d\"}],\"packageUris\":[\"http://schema.mathworks.com/mf0/Connector/R2020b\"],\"version\":\"1.0\"}"
  Raum4 : Subsystem
      settings: PortSchema="{\"entries\":[{\"content\":{\"sides\":[{\"content\":{\"connectorIds\":[\"Out1\",\"LConn1\",\"LConn2\"]},\"type\":\"ConnectorPlacement.EquallySpacedRectSide\",\"uuid\":\"258852ae-79b4-4e90-ae22-4154c858ab0a\"},{\"content\":{\"connectorIds\":[\"RConn1\"],\"side\":\"RIGHT\"},\"type\":\"ConnectorPlacement.EquallySpacedRectSide\",\"uuid\":\"36706832-f330-42ce-9a32-f145cdee4912\"},{\"content\":{\"connectorIds\":[\"LConn3\",\"LConn4\",\"LConn5\"],\"side\":\"TOP\"},\"type\":\"ConnectorPlacement.EquallySpacedRectSide\",\"uuid\":\"5cf2347a-3520-447e-9561-2d1c8313f3cf\"},{\"content\":{\"connectorIds\":[\"In1\",\"In2\",\"RConn2\"],\"side\":\"BOTTOM\"},\"type\":\"ConnectorPlacement.EquallySpacedRectSide\",\"uuid\":\"b1588268-8d41-4423-8f6e-2c28bf9b13dc\"}]},\"type\":\"ConnectorPlacement.EquallySpacedConnector\",\"uuid\":\"6bed35e7-1d7a-421b-a1f8-39267ed9017d\"}],\"packageUris\":[\"http://schema.mathworks.com/mf0/Connector/R2020b\"],\"version\":\"1.0\"}"
  Raum5 : Subsystem
      settings: PortSchema="{\"entries\":[{\"content\":{\"sides\":[{\"content\":{\"connectorIds\":[\"LConn1\",\"LConn2\",\"LConn3\"]},\"type\":\"ConnectorPlacement.EquallySpacedRectSide\",\"uuid\":\"258852ae-79b4-4e90-ae22-4154c858ab0a\"},{\"content\":{\"connectorIds\":[\"In2\"],\"side\":\"RIGHT\"},\"type\":\"ConnectorPlacement.EquallySpacedRectSide\",\"uuid\":\"36706832-f330-42ce-9a32-f145cdee4912\"},{\"content\":{\"connectorIds\":[\"LConn4\",\"Out1\"],\"side\":\"TOP\"},\"type\":\"ConnectorPlacement.EquallySpacedRectSide\",\"uuid\":\"5cf2347a-3520-447e-9561-2d1c8313f3cf\"},{\"content\":{\"connectorIds\":[\"RConn1\",\"In1\",\"RConn2\",\"RConn3\"],\"side\":\"BOTTOM\"},\"type\":\"ConnectorPlacement.EquallySpacedRectSide\",\"uuid\":\"b1588268-8d41-4423-8f6e-2c28bf9b13dc\"}]},\"type\":\"ConnectorPlacement.EquallySpacedConnector\",\"uuid\":\"6bed35e7-1d7a-421b-a1f8-39267ed9017d\"}],\"packageUris\":[\"http://schema.mathworks.com/mf0/Connector/R2020b\"],\"version\":\"1.0\"}"
  Raum6 : Subsystem
      settings: PortSchema="{\"entries\":[{\"content\":{\"sides\":[{\"content\":{\"connectorIds\":[\"LConn1\",\"LConn2\",\"LConn3\",\"LConn4\"]},\"type\":\"ConnectorPlacement.EquallySpacedRectSide\",\"uuid\":\"258852ae-79b4-4e90-ae22-4154c858ab0a\"},{\"content\":{\"connectorIds\":[\"Out1\"],\"side\":\"RIGHT\"},\"type\":\"ConnectorPlacement.EquallySpacedRectSide\",\"uuid\":\"36706832-f330-42ce-9a32-f145cdee4912\"},{\"content\":{\"connectorIds\":[\"LConn5\",\"LConn6\"],\"side\":\"TOP\"},\"type\":\"ConnectorPlacement.EquallySpacedRectSide\",\"uuid\":\"5cf2347a-3520-447e-9561-2d1c8313f3cf\"},{\"content\":{\"connectorIds\":[\"In1\",\"In2\",\"RConn1\"],\"side\":\"BOTTOM\"},\"type\":\"ConnectorPlacement.EquallySpacedRectSide\",\"uuid\":\"b1588268-8d41-4423-8f6e-2c28bf9b13dc\"}]},\"type\":\"ConnectorPlacement.EquallySpacedConnector\",\"uuid\":\"6bed35e7-1d7a-421b-a1f8-39267ed9017d\"}],\"packageUris\":[\"http://schema.mathworks.com/mf0/Connector/R2020b\"],\"version\":\"1.0\"}"
  Raum7 : Subsystem
      settings: PortSchema="{\"entries\":[{\"content\":{\"sides\":[{\"content\":{\"connectorIds\":[\"In1\",\"LConn1\",\"LConn2\"]},\"type\":\"ConnectorPlacement.EquallySpacedRectSide\",\"uuid\":\"258852ae-79b4-4e90-ae22-4154c858ab0a\"},{\"content\":{\"connectorIds\":[\"RConn1\",\"RConn2\",\"RConn3\"],\"side\":\"RIGHT\"},\"type\":\"ConnectorPlacement.EquallySpacedRectSide\",\"uuid\":\"36706832-f330-42ce-9a32-f145cdee4912\"},{\"content\":{\"connectorIds\":[\"LConn3\",\"LConn4\",\"LConn5\",\"Out1\",\"LConn6\",\"LConn7\"],\"side\":\"TOP\"},\"type\":\"ConnectorPlacement.EquallySpacedRectSide\",\"uuid\":\"5cf2347a-3520-447e-9561-2d1c8313f3cf\"},{\"content\":{\"connectorIds\":[\"RConn4\",\"RConn5\",\"RConn6\",\"In2\",\"RConn7\",\"RConn8\"],\"side\":\"BOTTOM\"},\"type\":\"ConnectorPlacement.EquallySpacedRectSide\",\"uuid\":\"b1588268-8d41-4423-8f6e-2c28bf9b13dc\"}]},\"type\":\"ConnectorPlacement.EquallySpacedConnector\",\"uuid\":\"6bed35e7-1d7a-421b-a1f8-39267ed9017d\"}],\"packageUris\":[\"http://schema.mathworks.com/mf0/Connector/R2020b\"],\"version\":\"1.0\"}"
  Raum8 : Subsystem
      settings: PortSchema="{\"entries\":[{\"content\":{\"sides\":[{\"content\":{\"connectorIds\":[\"LConn1\",\"Out1\",\"In1\"]},\"type\":\"ConnectorPlacement.EquallySpacedRectSide\",\"uuid\":\"258852ae-79b4-4e90-ae22-4154c858ab0a\"},{\"content\":{\"connectorIds\":[\"RConn1\",\"RConn2\"],\"side\":\"RIGHT\"},\"type\":\"ConnectorPlacement.EquallySpacedRectSide\",\"uuid\":\"36706832-f330-42ce-9a32-f145cdee4912\"},{\"content\":{\"connectorIds\":[\"LConn2\",\"LConn3\",\"LConn4\",\"LConn5\"],\"side\":\"TOP\"},\"type\":\"ConnectorPlacement.EquallySpacedRectSide\",\"uuid\":\"5cf2347a-3520-447e-9561-2d1c8313f3cf\"},{\"content\":{\"connectorIds\":[\"In2\"],\"side\":\"BOTTOM\"},\"type\":\"ConnectorPlacement.EquallySpacedRectSide\",\"uuid\":\"b1588268-8d41-4423-8f6e-2c28bf9b13dc\"}]},\"type\":\"ConnectorPlacement.EquallySpacedConnector\",\"uuid\":\"6bed35e7-1d7a-421b-a1f8-39267ed9017d\"}],\"packageUris\":[\"http://schema.mathworks.com/mf0/Connector/R2020b\"],\"version\":\"1.0\"}"
  Raum9 : Subsystem
      settings: PortSchema="{\"entries\":[{\"content\":{\"sides\":[{\"content\":{\"connectorIds\":[\"LConn1\",\"LConn2\",\"In1\"]},\"type\":\"ConnectorPlacement.EquallySpacedRectSide\",\"uuid\":\"258852ae-79b4-4e90-ae22-4154c858ab0a\"},{\"content\":{\"side\":\"RIGHT\"},\"type\":\"ConnectorPlacement.EquallySpacedRectSide\",\"uuid\":\"36706832-f330-42ce-9a32-f145cdee4912\"},{\"content\":{\"connectorIds\":[\"LConn3\",\"In2\",\"Out1\",\"LConn4\"],\"side\":\"TOP\"},\"type\":\"ConnectorPlacement.EquallySpacedRectSide\",\"uuid\":\"5cf2347a-3520-447e-9561-2d1c8313f3cf\"},{\"content\":{\"connectorIds\":[\"RConn1\",\"RConn2\",\"RConn3\"],\"side\":\"BOTTOM\"},\"type\":\"ConnectorPlacement.EquallySpacedRectSide\",\"uuid\":\"b1588268-8d41-4423-8f6e-2c28bf9b13dc\"}]},\"type\":\"ConnectorPlacement.EquallySpacedConnector\",\"uuid\":\"6bed35e7-1d7a-421b-a1f8-39267ed9017d\"}],\"packageUris\":[\"http://schema.mathworks.com/mf0/Connector/R2020b\"],\"version\":\"1.0\"}"
  Tatm12 : Sin  Amplitude=7  Frequency=2*pi/(24*3600)  Phase=pi  SampleTime=0
  pipe to 3 : Subsystem
  hot water in : PMIOPort  Side=Left
  Hot Water Out1 : PMIOPort  Port=2  Side=Right
  Y-6 Flur12OG2 : PMIOPort  Port=3  Side=Right
  Y-Flur11OG2 : PMIOPort  Port=4  Side=Right
  Y-Flur10OG2 : PMIOPort  Port=5  Side=Right
  Y-Flur9OG2 : PMIOPort  Port=6  Side=Right
  Y-Flur8OG2 : PMIOPort  Port=7  Side=Right
  Y-Flur7OG2 : PMIOPort  Port=8  Side=Right
  Y-Flur6OG2 : PMIOPort  Port=9  Side=Right
  Y-Flur5OG2 : PMIOPort  Port=10  Side=Right
  Y-Flur4OG2 : PMIOPort  Port=11  Side=Right
  Y-Flur3OG2 : PMIOPort  Port=12  Side=Right
  Y-Flur2OG2 : PMIOPort  Port=13  Side=Right
  Y-Flur1OG2 : PMIOPort  Port=14  Side=Right
  TroomOG2 : Outport
  wires:
  Raum9/1(Troom) -> [Traum9]
  [Traum4] -> Mux/4
  [Traum10] -> Mux/10
  [Tatm] -> Raum11/1(Tatm)
  Raum6/1(Troom) -> [Traum6]
  [Traum5] -> Mux/5
  [Traum7] -> Mux/7
  [Tatm] -> Raum9/1(Tatm)
  Raum7/1(Troom) -> [Traum7]
  [Traum9] -> Mux/9
  [Tatm] -> Raum7/1(Tatm)
  [Traum12] -> Mux/12
  Raum11/1(Troom) -> [Troom11]
  [Traum6] -> Mux/6
  [Tatm] -> Raum2/2(Tatm)
  Raum2/1(Troom) -> [Traum2]
  [Tatm] -> Raum10/1(Tatm)
  [Tatm] -> Raum1/1(Tatm)
  [Tatm] -> Raum5/2(Tatm)
  [Tatm] -> Raum3/2(Tatm)
  [Traum1] -> Mux/1
  [Tatm] -> Raum4/2(Tatm)
  [Traum2] -> Mux/2
  Raum10/1(Troom) -> [Traum10]
  Raum1/1(Troom) -> [Traum1]
  [Tatm] -> Raum6/1(Tatm)
  [Traum3] -> Mux/3
  [Tatm] -> Raum8/1(Tatm)
  Raum4/1(Troom) -> [Traum4]
  Raum5/1(Troom) -> [Traum5]
  [Traum8] -> Mux/8
  [Troom11] -> Mux/11
  Raum8/1(Troom) -> [Traum8]
  Raum12/1(Troom) -> [Traum12]
  [Tatm] -> Raum12/1(Tatm)
  Tatm12/1 -> [Tatm]
  Raum3/1(Troom) -> [Traum3]
  In1/1 -> Raum12/2(In2)
  In2/1 -> Raum2/1(In1)
  In3/1 -> Raum3/1(valve command)
  In4/1 -> Raum4/1(valve command)
  In5/1 -> Raum8/2(valve command)
  In6/1 -> Raum6/2(valve command)
  In7/1 -> Raum5/1(valve command)
  In10/1 -> Raum7/2(valve command)
  In11/1 -> Raum11/2(valve command)
  In9/1 -> Raum10/2(valve command)
  In8/1 -> Raum9/2(valve command)
  Mux/1 -> TroomOG2/1
  connections:
  Raum6/LConn4 -- Raum8/RConn2
  Raum3/LConn2 -- Raum4/RConn2 -- Hot Water Out1/RConn1 -- Raum5/RConn3 -- Raum6/RConn1 -- Raum8/LConn1 -- Raum10/LConn2 -- Raum9/LConn1 -- Raum11/LConn1 -- Raum7/RConn4 -- Raum2/LConn3 -- Raum12/LConn2
  Raum5/RConn2 -- Raum6/LConn6
  Raum7/RConn7 -- Raum6/LConn2
  Pipe to 6/RConn1 -- Raum6/LConn5
  Raum1/RConn2 -- Raum2/RConn4
  Pipe to 12/RConn1 -- Raum12/LConn1
  Pipe to 7/RConn1 -- Raum7/LConn3
  Raum11/LConn2 -- Raum12/RConn1
  Raum3/LConn4 -- Raum2/LConn4
  Raum4/LConn4 -- Raum2/RConn6
  Raum11/RConn4 -- Raum1/LConn4
  Raum9/LConn3 -- Pipe to 9a/RConn1
  Raum5/LConn4 -- Raum9/RConn3
  Pipe to 4/RConn1 -- Raum4/LConn1
  Raum7/RConn8 -- Raum6/LConn1
  Pipe to 8/RConn1 -- Raum8/LConn3
  Pipe to 11/RConn1 -- Raum11/LConn3
  Raum9/RConn2 -- Raum7/RConn1
  Raum10/LConn1 -- Raum11/RConn1
  Raum2/LConn6 -- Raum12/RConn4
  Raum7/LConn2 -- Raum1/LConn3
  Pipe to 10/RConn1 -- Raum10/LConn4
  pipe to 3/RConn1 -- Raum3/LConn1
  Raum1/RConn3 -- Raum8/LConn2
  Raum9/LConn2 -- Raum10/RConn1
  Raum5/LConn3 -- Raum7/RConn3
  Raum2/RConn5 -- Raum4/LConn3
  Raum7/RConn5 -- Raum8/LConn4
  Raum3/LConn3 -- Raum12/RConn2
  Raum10/LConn3 -- Raum1/LConn1
  Pipe to 2/RConn1 -- Raum2/LConn2
  Raum12/RConn3 -- Raum2/LConn5
  Raum10/RConn3 -- Raum7/LConn5
  Raum7/RConn2 -- Raum5/LConn2
  Raum11/RConn2 -- Raum2/RConn2
  Raum3/LConn5 -- Raum2/LConn1
  Raum9/RConn1 -- Raum7/LConn6
  Raum3/RConn1 -- Raum4/LConn2
  Pipe to 5/RConn1 -- Raum5/RConn1
  Raum1/RConn4 -- Raum4/RConn1
  Raum1/LConn2 -- Raum7/LConn1
  Raum11/RConn3 -- Raum2/RConn3
  Raum8/LConn5 -- Raum7/RConn6
  Raum7/LConn4 -- Raum10/RConn2
  Raum2/RConn1 -- Raum1/RConn1
  Raum12/LConn3 -- Y-6 Flur12OG2/RConn1
  Raum11/LConn4 -- Y-Flur11OG2/RConn1
  Raum10/LConn5 -- Y-Flur10OG2/RConn1
  Raum9/LConn4 -- Y-Flur9OG2/RConn1
  Y-Flur5OG2/RConn1 -- Raum5/LConn1
  Raum7/LConn7 -- Y-Flur7OG2/RConn1
  Y-Flur6OG2/RConn1 -- Raum6/LConn3
  Y-Flur8OG2/RConn1 -- Raum8/RConn1
  Raum1/LConn5 -- Y-Flur1OG2/RConn1
  Y-Flur4OG2/RConn1 -- Raum4/LConn5
  Raum3/RConn2 -- Y-Flur3OG2/RConn1
  Raum2/LConn7 -- Y-Flur2OG2/RConn1
  hot water in/RConn1 -- Pipe to 4/LConn1 -- Pipe to 12/LConn1 -- Pipe to 7/LConn1 -- Pipe to 8/LConn1 -- Pipe to 6/LConn1 -- Pipe to 5/LConn1 -- Pipe to 9a/LConn1 -- Pipe to 10/LConn1 -- Pipe to 11/LConn1 -- Pipe to 2/LConn1 -- pipe to 3/LConn1

== system Main_SpeedOptimisedVersionTannenweg/Pump ==
  Centrifugal Pump (TL) : SimscapeFluids_lib/Thermal Liquid/Pumps & Motors/Centrifugal Pump (TL)  pump_parameterization=fluids.thermal_liquid.pumps_motors.enum.CentrifugalPumpParameterization.Table1D  capacity_ref_nominal=45 lpm  head_ref_nominal=40 m  power_ref_nominal=0.85 kW  head_ref_max=60 m  capacity_ref_max=80 lpm  omega_ref_analytic=1770 rpm  flow_rate_1D_TLU=[16.67, 30, 40, 53.33, 66.67, 83.33] lpm  head_1D_TLU=[50, 47.5, 45, 40, 35, 25] m  power_1D_TLU=[.6, .75, .85, .93, .98, .99] kW  omega_ref_1D=3500 rpm  rho_ref_1D=998.21 kg/m^3  omega_threshold_factor=1e-2  flow_rate_2D_TLU=[16.67, 23.33, 30, 40, 53.33, 60] lpm  omega_2D_TLU=[2450, 2800, 3150, 3500] rpm  head_2D_TLU=[25, 32.7, 42.5, 50; 24, 31.7, 41, 49; 22.7, 30.5, 39, 47.5; 20, 28, 36, 45; 15.7, 24, 32, 40; 12.5, 21, 29.5, 37.5] m  power_2D_TLU=[.28, .38, .5, .6; .31, .41, .55, .68; .33, .44, .6, .75; .36, .48, .65, .83; .38, .53, .72, .93; .39, .55, .75, .97] kW  rho_ref_2D=998.21 kg/m^3  diameter_ratio=1  mech_orientation=fluids.thermal_liquid.pumps_motors.enum.CentrifugalPumpMechOrientation.Positive  area=ma m^2  operation_check=simscape.enum.assert.action.none
      settings: InternalSimscapePortConfiguration="{\"Bottom\":[],\"Left\":[{\"id\":\"A\",\"label\":\"A\",\"type\":\"foundation.thermal_liquid.thermal_liquid\"},{\"id\":\"B\",\"label\":\"B\",\"type\":\"foundation.thermal_liquid.thermal_liquid\"}],\"Right\":[{\"id\":\"R\",\"label\":\"R\",\"type\":\"foundation.mechanical.rotational.rotational\"},{\"id\":\"C\",\"label\":\"C\",\"type\":\"foundation.mechanical.rotational.rotational\"}],\"Top\":[]}"
  Constant : Constant  Value=100
  Ideal Angular Velocity Source : fl_lib/Mechanical/Mechanical Sources/Ideal Angular Velocity Source
  Mechanical Rotational Reference : fl_lib/Mechanical/Rotational Elements/Mechanical Rotational Reference
  Simulink-PS Converter1 : nesl_utility/Simulink-PS Converter  PhysicalDomain=network_engine_domain  SubClassName=ps_input  LeftPortType=input  RightPortType=output  PseudoPeriodic=off  Frequencies=[]  NoiseDistribution=none  NoiseParameters=[]  Unit=1  AffineConversion=off  FilteringAndDerivatives=provide  SimscapeFilterOrder=1  InputFilterTimeConstant=0.001  UdotUserProvided=0
  OUT : PMIOPort  Side=Left
  IN : PMIOPort  Port=2  Side=Right
  wires:
  Constant/1 -> Simulink-PS Converter1/1
  connections:
  Ideal Angular Velocity Source/RConn2 -- Centrifugal Pump (TL)/RConn2 -- Mechanical Rotational Reference/LConn1
  IN/RConn1 -- Centrifugal Pump (TL)/LConn1
  Centrifugal Pump (TL)/LConn2 -- OUT/RConn1
  Ideal Angular Velocity Source/LConn1 -- Centrifugal Pump (TL)/RConn1
  Simulink-PS Converter1/RConn1 -- Ideal Angular Velocity Source/RConn1

== system Main_SpeedOptimisedVersionTannenweg/Subsystem Boiler Controller ==
  Heat Input : Inport
  Constant : Constant  Value=-1
  Constant1 : Constant  Value=-273.15
  Controlled Heat Flow Rate Source : fl_lib/Thermal/Thermal Sources/Controlled Heat Flow Rate Source
  Controller Relay : Relay  OnSwitchValue=-305  OffSwitchValue=-308  OffOutputValue=0.008
  Memory : Memory
  PS-Simulink Converter : nesl_utility/PS-Simulink Converter  PhysicalDomain=network_engine_domain  SubClassName=ps_output  LeftPortType=input  RightPortType=output  PseudoPeriodic=off  Frequencies=[]  VectorFormat=inherit  Unit=inherit  AffineConversion=off
  Product : Product
  Product1 : Product
  Simulink-PS Converter : nesl_utility/Simulink-PS Converter  PhysicalDomain=network_engine_domain  SubClassName=ps_input  LeftPortType=input  RightPortType=output  PseudoPeriodic=off  Frequencies=[]  NoiseDistribution=none  NoiseParameters=[]  Unit=1  AffineConversion=off  FilteringAndDerivatives=provide  SimscapeFilterOrder=1  InputFilterTimeConstant=0.001  UdotUserProvided=0
  Sum : Sum  Inputs=|++
  Thermal Reference : fl_lib/Thermal/Thermal Elements/Thermal Reference
  Heat supply to tank : PMIOPort  Side=Left
  hot water temp : PMIOPort  Port=2  Side=Left
  Output : Outport
  wires:
  Product/1 -> Controller Relay/1
  Constant/1 -> Product/2
  Product1/1 -> Simulink-PS Converter/1
  Heat Input/1 -> Product1/1
  PS-Simulink Converter/1 -> Sum/1, Memory/1
  Controller Relay/1 -> Product1/2
  Memory/1 -> Product/1
  Constant1/1 -> Sum/2
  Sum/1 -> Output/1
  connections:
  Simulink-PS Converter/RConn1 -- Controlled Heat Flow Rate Source/RConn1
  Thermal Reference/LConn1 -- Controlled Heat Flow Rate Source/RConn2
  Controlled Heat Flow Rate Source/LConn1 -- Heat supply to tank/RConn1
  hot water temp/RConn1 -- PS-Simulink Converter/LConn1

== system Main_SpeedOptimisedVersionTannenweg/EG/Pipe to 10 ==
  Perfect Insulator3 : fl_lib/Thermal/Thermal Elements/Perfect Insulator  T_specify=off  T_priority=None  T=293.15 K  T_nominal_specify=off  T_nominal_value=1  T_nominal_unit=K
  Pipe (TL)3 : fl_lib/Thermal Liquid/Elements/Pipe (TL)  length=5.88 m  area=fa m^2  Dh=fd m  length_add=1 m  roughness=15e-6 m  Re_lam=2000  Re_tur=4000  shape_factor=64  Nu_lam=3.66  dynamic_compressibility=true  inertia=false  p0=0.101325 MPa  T0=293.15 K  mdot0=0 kg/s
  out : PMIOPort  Side=Right
  in : PMIOPort  Port=2  Side=Left
  connections:
  Perfect Insulator3/LConn1 -- Pipe (TL)3/LConn2
  in/RConn1 -- Pipe (TL)3/LConn1
  Pipe (TL)3/RConn1 -- out/RConn1

== system Main_SpeedOptimisedVersionTannenweg/EG/Pipe to 11 ==
  Perfect Insulator3 : fl_lib/Thermal/Thermal Elements/Perfect Insulator  T_specify=off  T_priority=None  T=293.15 K  T_nominal_specify=off  T_nominal_value=1  T_nominal_unit=K
  Pipe (TL)3 : fl_lib/Thermal Liquid/Elements/Pipe (TL)  length=5.32 m  area=fa m^2  Dh=fd m  length_add=1 m  roughness=15e-6 m  Re_lam=2000  Re_tur=4000  shape_factor=64  Nu_lam=3.66  dynamic_compressibility=true  inertia=false  p0=0.101325 MPa  T0=293.15 K  mdot0=0 kg/s
  out : PMIOPort  Side=Right
  in : PMIOPort  Port=2  Side=Left
  connections:
  in/RConn1 -- Pipe (TL)3/LConn1
  Perfect Insulator3/LConn1 -- Pipe (TL)3/LConn2
  Pipe (TL)3/RConn1 -- out/RConn1

== system Main_SpeedOptimisedVersionTannenweg/EG/Pipe to 12 ==
  Perfect Insulator3 : fl_lib/Thermal/Thermal Elements/Perfect Insulator  T_specify=off  T_priority=None  T=293.15 K  T_nominal_specify=off  T_nominal_value=1  T_nominal_unit=K
  Pipe (TL)3 : fl_lib/Thermal Liquid/Elements/Pipe (TL)  length=7.7 m  area=fa m^2  Dh=fd m  length_add=1 m  roughness=15e-6 m  Re_lam=2000  Re_tur=4000  shape_factor=64  Nu_lam=3.66  dynamic_compressibility=true  inertia=false  p0=0.101325 MPa  T0=293.15 K  mdot0=0 kg/s
  out : PMIOPort  Side=Right
  in : PMIOPort  Port=2  Side=Left
  connections:
  Perfect Insulator3/LConn1 -- Pipe (TL)3/LConn2
  in/RConn1 -- Pipe (TL)3/LConn1
  Pipe (TL)3/RConn1 -- out/RConn1

== system Main_SpeedOptimisedVersionTannenweg/EG/Pipe to 2 ==
  Perfect Insulator1 : fl_lib/Thermal/Thermal Elements/Perfect Insulator  T_specify=off  T_priority=None  T=293.15 K  T_nominal_specify=off  T_nominal_value=1  T_nominal_unit=K
  Pipe (TL)1 : fl_lib/Thermal Liquid/Elements/Pipe (TL)  length=2.38 m  area=fa m^2  Dh=fd m  length_add=1 m  roughness=15e-6 m  Re_lam=2000  Re_tur=4000  shape_factor=64  Nu_lam=3.66  dynamic_compressibility=true  inertia=false  p0=0.101325 MPa  T0=293.15 K  mdot0=0 kg/s
  Conn1 : PMIOPort  Side=Left
  Conn2 : PMIOPort  Port=2  Side=Right
  connections:
  Pipe (TL)1/RConn1 -- Conn2/RConn1
  Perfect Insulator1/LConn1 -- Pipe (TL)1/LConn2
  Conn1/RConn1 -- Pipe (TL)1/LConn1

== system Main_SpeedOptimisedVersionTannenweg/EG/Pipe to 4 ==
  Perfect Insulator2 : fl_lib/Thermal/Thermal Elements/Perfect Insulator  T_specify=off  T_priority=None  T=293.15 K  T_nominal_specify=off  T_nominal_value=1  T_nominal_unit=K
  Pipe (TL)2 : fl_lib/Thermal Liquid/Elements/Pipe (TL)  length=7.38 m  area=fa m^2  Dh=fd m  length_add=1 m  roughness=15e-6 m  Re_lam=2000  Re_tur=4000  shape_factor=64  Nu_lam=3.66  dynamic_compressibility=true  inertia=false  p0=0.101325 MPa  T0=293.15 K  mdot0=0 kg/s
  in : PMIOPort  Side=Left
  out : PMIOPort  Port=2  Side=Right
  connections:
  Perfect Insulator2/LConn1 -- Pipe (TL)2/LConn2
  Pipe (TL)2/LConn1 -- in/RConn1
  Pipe (TL)2/RConn1 -- out/RConn1

== system Main_SpeedOptimisedVersionTannenweg/EG/Pipe to 5 ==
  Perfect Insulator3 : fl_lib/Thermal/Thermal Elements/Perfect Insulator  T_specify=off  T_priority=None  T=293.15 K  T_nominal_specify=off  T_nominal_value=1  T_nominal_unit=K
  Pipe (TL)3 : fl_lib/Thermal Liquid/Elements/Pipe (TL)  length=12.42 m  area=fa m^2  Dh=fd m  length_add=1 m  roughness=15e-6 m  Re_lam=2000  Re_tur=4000  shape_factor=64  Nu_lam=3.66  dynamic_compressibility=true  inertia=false  p0=0.101325 MPa  T0=293.15 K  mdot0=0 kg/s
  out : PMIOPort  Side=Right
  in : PMIOPort  Port=2  Side=Left
  connections:
  Perfect Insulator3/LConn1 -- Pipe (TL)3/LConn2
  Pipe (TL)3/RConn1 -- out/RConn1
  in/RConn1 -- Pipe (TL)3/LConn1

== system Main_SpeedOptimisedVersionTannenweg/EG/Pipe to 6 ==
  Perfect Insulator3 : fl_lib/Thermal/Thermal Elements/Perfect Insulator  T_specify=off  T_priority=None  T=293.15 K  T_nominal_specify=off  T_nominal_value=1  T_nominal_unit=K
  Pipe (TL)3 : fl_lib/Thermal Liquid/Elements/Pipe (TL)  length=9.34 m  area=fa m^2  Dh=fd m  length_add=1 m  roughness=15e-6 m  Re_lam=2000  Re_tur=4000  shape_factor=64  Nu_lam=3.66  dynamic_compressibility=true  inertia=false  p0=0.101325 MPa  T0=293.15 K  mdot0=0 kg/s
  out : PMIOPort  Side=Right
  in : PMIOPort  Port=2  Side=Left
  connections:
  in/RConn1 -- Pipe (TL)3/LConn1
  Perfect Insulator3/LConn1 -- Pipe (TL)3/LConn2
  Pipe (TL)3/RConn1 -- out/RConn1

== system Main_SpeedOptimisedVersionTannenweg/EG/Pipe to 7 ==
  Perfect Insulator3 : fl_lib/Thermal/Thermal Elements/Perfect Insulator  T_specify=off  T_priority=None  T=293.15 K  T_nominal_specify=off  T_nominal_value=1  T_nominal_unit=K
  Pipe (TL)3 : fl_lib/Thermal Liquid/Elements/Pipe (TL)  length=3.5 m  area=fa m^2  Dh=fd m  length_add=1 m  roughness=15e-6 m  Re_lam=2000  Re_tur=4000  shape_factor=64  Nu_lam=3.66  dynamic_compressibility=true  inertia=false  p0=0.101325 MPa  T0=293.15 K  mdot0=0 kg/s
  out : PMIOPort  Side=Right
  " in" : PMIOPort  Port=2  Side=Left
  connections:
  Perfect Insulator3/LConn1 -- Pipe (TL)3/LConn2
  " in"/RConn1 -- Pipe (TL)3/LConn1
  Pipe (TL)3/RConn1 -- out/RConn1

== system Main_SpeedOptimisedVersionTannenweg/EG/Pipe to 8 ==
  Perfect Insulator3 : fl_lib/Thermal/Thermal Elements/Perfect Insulator  T_specify=off  T_priority=None  T=293.15 K  T_nominal_specify=off  T_nominal_value=1  T_nominal_unit=K
  Pipe (TL)3 : fl_lib/Thermal Liquid/Elements/Pipe (TL)  length=10.04 m  area=fa m^2  Dh=fd m  length_add=1 m  roughness=15e-6 m  Re_lam=2000  Re_tur=4000  shape_factor=64  Nu_lam=3.66  dynamic_compressibility=true  inertia=false  p0=0.101325 MPa  T0=293.15 K  mdot0=0 kg/s
  out : PMIOPort  Side=Right
  in : PMIOPort  Port=2  Side=Left
  connections:
  Perfect Insulator3/LConn1 -- Pipe (TL)3/LConn2
  in/RConn1 -- Pipe (TL)3/LConn1
  Pipe (TL)3/RConn1 -- out/RConn1

== system Main_SpeedOptimisedVersionTannenweg/EG/Pipe to 9a ==
  Perfect Insulator3 : fl_lib/Thermal/Thermal Elements/Perfect Insulator  T_specify=off  T_priority=None  T=293.15 K  T_nominal_specify=off  T_nominal_value=1  T_nominal_unit=K
  Pipe (TL)3 : fl_lib/Thermal Liquid/Elements/Pipe (TL)  length=10.14 m  area=fa m^2  Dh=fd m  length_add=1 m  roughness=15e-6 m  Re_lam=2000  Re_tur=4000  shape_factor=64  Nu_lam=3.66  dynamic_compressibility=true  inertia=false  p0=0.101325 MPa  T0=293.15 K  mdot0=0 kg/s
  out : PMIOPort  Side=Right
  in : PMIOPort  Port=2  Side=Left
  connections:
  in/RConn1 -- Pipe (TL)3/LConn1
  Perfect Insulator3/LConn1 -- Pipe (TL)3/LConn2
  Pipe (TL)3/RConn1 -- out/RConn1
